simulink model "sf_while"  (R2025b)
settings: Solver=FixedStepDiscrete  StartTime=0.0  StopTime=1  FixedStep=1  RelTol=1e-3  EnableMultiTasking=on
settings Model: FPTRunName=Active  ExtModeAutoUpdateStatusClock=off  Creator=The MathWorks, Inc.  LastModifiedBy=The MathWorks, Inc.
settings SolverCC: AlgebraicLoopSolver=TrustRegion
settings DataIOCC: LimitDataPoints=on  SaveFormat=Array  ReturnWorkspaceOutputs=off  SignalLoggingName=sigsOut
settings OptimizationCC: ReuseModelBlockBuffer=off  ExpressionDepthLimit=2147483647.0  InitFltsAndDblsToZero=on  EfficientMapNaN2IntZero=off  LifeSpan=inf
settings DebuggingCC: SaveWithParameterizedLinksMsg=none  UnderspecifiedInitializationDetection=Classic  MergeDetectMultiDrivingBlocksExec=none  SignalResolutionControl=TryResolveAllWithWarning  MultiTaskDSMMsg=warning  MultiTaskCondExecSysMsg=none  FcnCallInpInsideContextMsg=warning  UnconnectedInputMsg=warning  UnconnectedOutputMsg=warning  UnconnectedLineMsg=warning  AllowSymbolicDim=off  StateNameClashWarn=warning  SFUnexpectedBacktrackingDiag=warning  SFNoUnconditionalDefaultTransitionDiag=warning  SFExecutionAtInitializationDiag=none  ArithmeticOperatorsInVariantConditions=warning
settings HardwareCC: ProdBitPerPointer=32.0  ProdBitPerSizeT=32.0  ProdBitPerPtrDiffT=32.0  ProdLargestAtomicFloat=None  ProdIntDivRoundTo=Undefined  ProdEndianess=Unspecified  ProdWordSize=32.0  ProdHWDeviceType=32-bit Generic  TargetUnknown=on
settings ModelReferenceCC: EnableRefExpFcnMdlSchedulingChecks=on  PropagateSignalLabelsOutOfModel=off
settings SFSimCC: SimUseLocalCustomCode=off  SimParseCustomCode=off  CustomCodeUndefinedFunction=UseInterfaceOnly
settings RTWCC: RTWUseLocalCustomCode=off  GPUComputeCapability=3.5
settings CodeAppCC: StateflowObjectComments=on
settings GRTTargetCC: TargetFcnLib=ansi_tfl_tmw.mat  TargetLangStandard=C89/C90 (ANSI)  CombineOutputUpdateFcns=off  GRTInterface=on
settings ConfigComp: CovMetricSettings=dcmtr  CovSaveCumulativeToWorkspaceVar=on  CovSaveSingleToWorkspaceVar=on  CovExternalEMLEnable=off  CovSFcnEnable=off

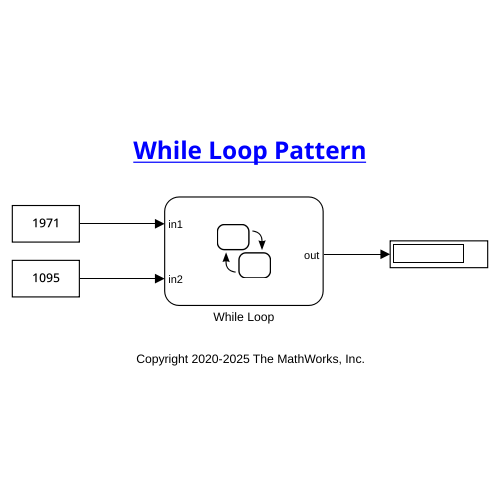
[thumbnail: Simulink's stored preview of the top-level diagram]
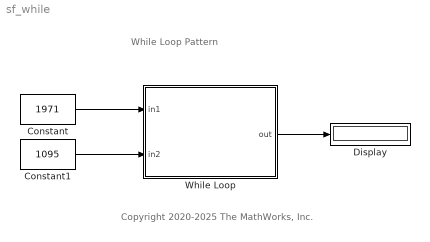
== system sf_while ==
  note: Copyright 2020-2025 The MathWorks, Inc.
  note: While Loop Pattern
  Constant : Constant  Value=1971
  Constant1 : Constant  Value=1095
  Display : Display
  While Loop : Stateflow chart  TreatAsAtomicUnit=on
  wires:
  While Loop/1(out) -> Display/1
  Constant/1 -> While Loop/1(in1)
  Constant1/1 -> While Loop/2(in2)

== stateflow chart sf_while/While Loop ==
  (default) -> (junction 40)
  (junction 40) -> (junction 32) : {
      |   p = max(in1,in2);
      |   q = min(in1,in2);
      | }
  (junction 32) -> (junction 31) [order 1] : [q > 0]
  (junction 33) -> (junction 32)
  (junction 32) -> (junction 34) [order 2] : {
      |   out = p;
      | }
  (junction 31) -> (junction 33) : {
      |   r = fmod(p,q);
      |   p = q;
      |   q = r;
      | }
  data: in1 input; out output double size=1; p local double; q local double; r local double; in2 input
